simulink model "radio_FM_simulink_final"  (R2026b)
settings: Solver=FixedStepDiscrete  StopTime=0.6  FixedStep=sampling_time
values from neighbouring files (symbols this model uses):
  DC_fm = G_dem*fc_fm/df    [parametros.m]
  df = beta*B_fdm    (= 6000)    [parametros.m]
  epsilon = 1e-8    (= 1e-08)    [parametros.m]
  fc_am2 = 400    [parametros.m]
  fc_am3 = 800    [parametros.m]
  fc_fm = evalin('base','fc_fm')    [radio_gui.m]
  flo = f_rx + fi    [parametros.m]
  G_fdm = 1/(3*(1+mu))    (= 0.222222222222)    [parametros.m]
  K_am = pi/(G_fdm*mu) / (1 + (select == 1))    [parametros.m]
  Kdem = G_dem/(4*df)    (= 5.25945833333e-05)    [parametros.m]
  mu = 0.5    [parametros.m]
  sampling_time = 2e-6    (= 2e-06)    [parametros.m]
  select = evalin('base','select')    [radio_gui.m]
  Ts_d = M*sampling_time    (= 1e-05)    [parametros.m]
undefined symbols (not defined in the file or in its folder): dfilt, DiscIntNeverNeededParam
libraries: dsparch4 x6, simulink x2, dspfdesign x2
settings Model: Creator=henao  LastModifiedBy=henao
settings DataIOCC: SaveOutput=off  SignalLogging=off

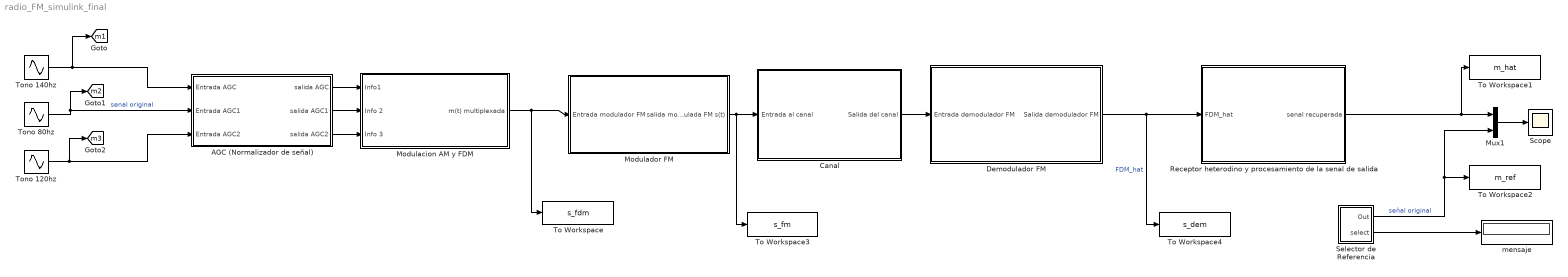
== system radio_FM_simulink_final ==
  AGC (Normalizador de señal) : Subsystem
  Canal : Subsystem
  Demodulador FM : Subsystem
  Modulacion AM y FDM : Subsystem
  Modulador FM : Subsystem
  Mux1 : Mux  Inputs=2
  Receptor heterodino y procesamiento de la senal de salida : Subsystem
  Scope : Scope
      settings: ActiveDisplayYMinimum=-1.3000748923673051  ActiveDisplayYMaximum=1.4483911176707998
  Selector de Referencia : Subsystem
  To Workspace : ToWorkspace  VariableName=s_fdm  SampleTime=-1
  To Workspace1 : ToWorkspace  VariableName=m_hat  SampleTime=-1
  To Workspace2 : ToWorkspace  VariableName=m_ref  SampleTime=-1
  To Workspace3 : ToWorkspace  VariableName=s_fm  SampleTime=-1
  To Workspace4 : ToWorkspace  VariableName=s_dem  SampleTime=-1
  Tono 120hz : Sin  Frequency=120*2*pi  SampleTime=sampling_time
  Tono 140hz : Sin  Amplitude=2  Frequency=140*2*pi  SampleTime=sampling_time
  Tono 80hz : Sin  Amplitude=3  Frequency=80*2*pi  SampleTime=sampling_time
  mensaje : Display
  tag scope: m1=global, m2=global, m3=global
  wires:
  Tono 80hz/1 -> AGC (Normalizador de señal)/2(Entrada AGC1), [m2]  "senal original"
  Tono 120hz/1 -> AGC (Normalizador de señal)/3(Entrada AGC2), [m3]
  Tono 140hz/1 -> AGC (Normalizador de señal)/1(Entrada AGC), [m1]
  AGC (Normalizador de señal)/1(salida AGC) -> Modulacion AM y FDM/1(Info1)
  AGC (Normalizador de señal)/2(salida AGC1) -> Modulacion AM y FDM/2(Info 2)
  AGC (Normalizador de señal)/3(salida AGC2) -> Modulacion AM y FDM/3(Info 3)
  Modulador FM/1(salida modulada FM s(t)) -> To Workspace3/1, Canal/1(Entrada al canal)
  Canal/1(Salida del canal) -> Demodulador FM/1(Entrada demodulador FM)
  Receptor heterodino y procesamiento de la senal de salida/1(senal recuperada) -> To Workspace1/1, Mux1/1
  Mux1/1 -> Scope/1
  Demodulador FM/1(Salida demodulador FM) -> To Workspace4/1, Receptor heterodino y procesamiento de la senal de salida/1(FDM_hat)  "FDM_hat"
  Selector de Referencia/1(Out) -> To Workspace2/1, Mux1/2  "señal original"
  Modulacion AM y FDM/1("m(t) multiplexada ") -> To Workspace/1, Modulador FM/1(Entrada modulador FM)
  Selector de Referencia/2(select) -> mensaje/1

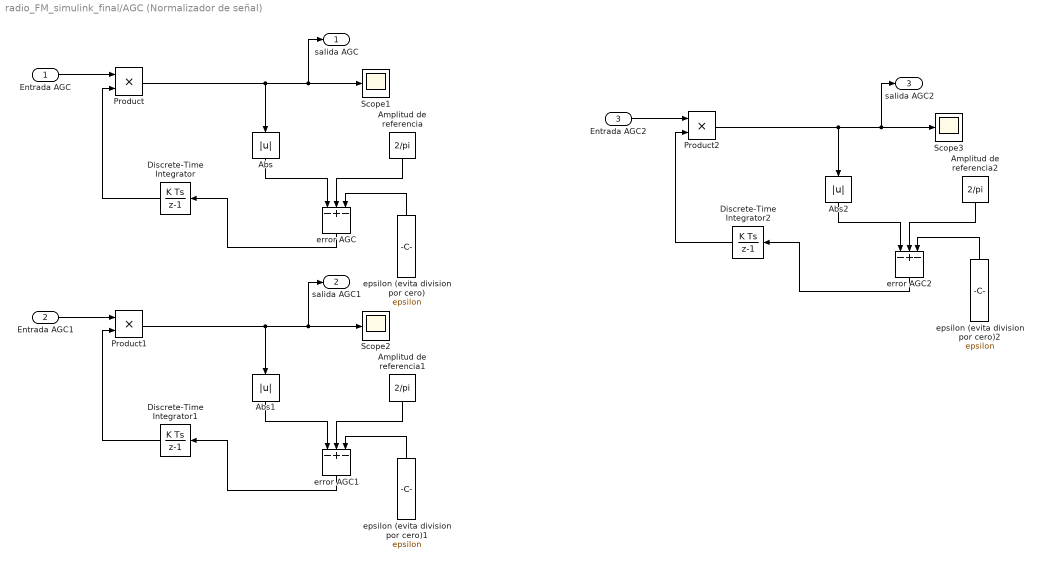
== system radio_FM_simulink_final/AGC (Normalizador de señal) ==
  Entrada AGC : Inport
  Entrada AGC1 : Inport  Port=2
  Entrada AGC2 : Inport  Port=3
  Abs : Abs  SaturateOnIntegerOverflow=off
  Abs1 : Abs  SaturateOnIntegerOverflow=off
  Abs2 : Abs  SaturateOnIntegerOverflow=off
  Amplitud de referencia : Constant  Value=2/pi
  Amplitud de referencia1 : Constant  Value=2/pi
  Amplitud de referencia2 : Constant  Value=2/pi
  Discrete-Time Integrator : DiscreteIntegrator  gainval=10  SampleTime=sampling_time  ICPrevOutput=DiscIntNeverNeededParam  ICPrevScaledInput=DiscIntNeverNeededParam
  Discrete-Time Integrator1 : DiscreteIntegrator  gainval=10  SampleTime=sampling_time  ICPrevOutput=DiscIntNeverNeededParam  ICPrevScaledInput=DiscIntNeverNeededParam
  Discrete-Time Integrator2 : DiscreteIntegrator  gainval=10  SampleTime=sampling_time  ICPrevOutput=DiscIntNeverNeededParam  ICPrevScaledInput=DiscIntNeverNeededParam
  Product : Product
  Product1 : Product
  Product2 : Product
  Scope1 : Scope
      settings: ActiveDisplayYMinimum=-1.05206  ActiveDisplayYMaximum=1.11653  DataLoggingVariableName=ScopeData3
  Scope2 : Scope
      settings: ActiveDisplayYMinimum=-1.05206  ActiveDisplayYMaximum=1.11653  DataLoggingVariableName=ScopeData2
  Scope3 : Scope
      settings: ActiveDisplayYMinimum=-1.05206  ActiveDisplayYMaximum=1.11653  DataLoggingVariableName=ScopeData4
  epsilon (evita division por cero) : Constant  Value=epsilon
  epsilon (evita division por cero)1 : Constant  Value=epsilon
  epsilon (evita division por cero)2 : Constant  Value=epsilon
  error AGC : Sum  Inputs=-+-
  error AGC1 : Sum  Inputs=-+-
  error AGC2 : Sum  Inputs=-+-
  salida AGC : Outport
  salida AGC1 : Outport  Port=2
  salida AGC2 : Outport  Port=3
  wires:
  error AGC/1 -> Discrete-Time Integrator/1
  Product/1 -> Abs/1, salida AGC/1, Scope1/1
  Abs/1 -> error AGC/1
  Amplitud de referencia/1 -> error AGC/2
  epsilon (evita division por cero)/1 -> error AGC/3
  Discrete-Time Integrator/1 -> Product/2
  Entrada AGC/1 -> Product/1
  Abs1/1 -> error AGC1/1
  Product1/1 -> Abs1/1, salida AGC1/1, Scope2/1
  epsilon (evita division por cero)1/1 -> error AGC1/3
  Entrada AGC1/1 -> Product1/1
  Amplitud de referencia1/1 -> error AGC1/2
  Discrete-Time Integrator1/1 -> Product1/2
  error AGC1/1 -> Discrete-Time Integrator1/1
  epsilon (evita division por cero)2/1 -> error AGC2/3
  error AGC2/1 -> Discrete-Time Integrator2/1
  Amplitud de referencia2/1 -> error AGC2/2
  Product2/1 -> Abs2/1, salida AGC2/1, Scope3/1
  Entrada AGC2/1 -> Product2/1
  Abs2/1 -> error AGC2/1
  Discrete-Time Integrator2/1 -> Product2/2

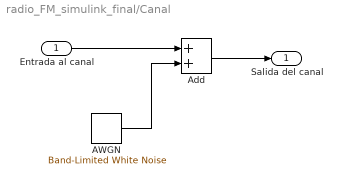
== system radio_FM_simulink_final/Canal ==
  Entrada al canal : Inport
  AWGN : simulink/Sources/Band-Limited White Noise  Cov=sigma2  Ts=sampling_time  seed=seed_ruido
  Add : Sum
  Salida del canal : Outport
  wires:
  Add/1 -> Salida del canal/1
  Entrada al canal/1 -> Add/1
  AWGN/1 -> Add/2

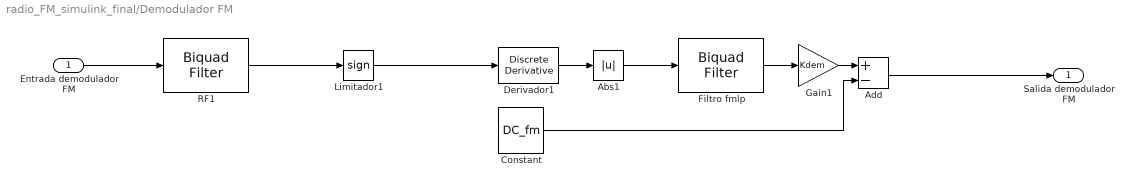
== system radio_FM_simulink_final/Demodulador FM ==
  Entrada demodulador FM : Inport
  Abs1 : Abs  SaturateOnIntegerOverflow=off
  Add : Sum  Inputs=+-
  Constant : Constant  Value=DC_fm
  Derivador1 : simulink/Discrete/Discrete Derivative  gainval=1  ICPrevScaledInput=0.0  OutMin=[]  OutMax=[]  OutDataType=fixdt(1, 16)  OutScaling=2^-10  DoSatur=off
  Filtro fmlp : dsparch4/Biquad Filter  FilterSource=Dialog parameters  CoeffSource=Specify via dialog  FilterObject=dfilt.df2tsos([1 0.3 0.4],[1 0.1 0.2])  IIRFiltStruct=Direct form II transposed  BiQuadCoeffs=sos_fmlp  ScaleValues=1  IC=0  ICnum=0  ICden=0  a0Flag=Warning  optimizeScaleValues=on  ScaleValueMode=Specify via input port (g)  roundingMode=Floor  overflowMode=off  scaleValueFracLength=14  denProdOutputFracLength=30  denAccumFracLength=30  secondMemoryFracLength=15
      settings: LibrarySourceBlock=dsphdlsupportfiltering/Biquad Filter
  Gain1 : Gain  Gain=Kdem
  Limitador1 : Signum
  RF1 : dsparch4/Biquad Filter  FilterSource=Dialog parameters  CoeffSource=Specify via dialog  FilterObject=dfilt.df2tsos([1 0.3 0.4],[1 0.1 0.2])  IIRFiltStruct=Direct form II transposed  BiQuadCoeffs=sos_rf  ScaleValues=1  IC=0  ICnum=0  ICden=0  a0Flag=Warning  optimizeScaleValues=on  ScaleValueMode=Specify via input port (g)  roundingMode=Floor  overflowMode=off  scaleValueFracLength=14  denProdOutputFracLength=30  denAccumFracLength=30  secondMemoryFracLength=15
      settings: LibrarySourceBlock=dsphdlsupportfiltering/Biquad Filter
  Salida demodulador FM : Outport
  wires:
  Entrada demodulador FM/1 -> RF1/1
  Filtro fmlp/1 -> Gain1/1
  Abs1/1 -> Filtro fmlp/1
  Derivador1/1 -> Abs1/1
  Limitador1/1 -> Derivador1/1
  RF1/1 -> Limitador1/1
  Add/1 -> Salida demodulador FM/1
  Gain1/1 -> Add/1
  Constant/1 -> Add/2

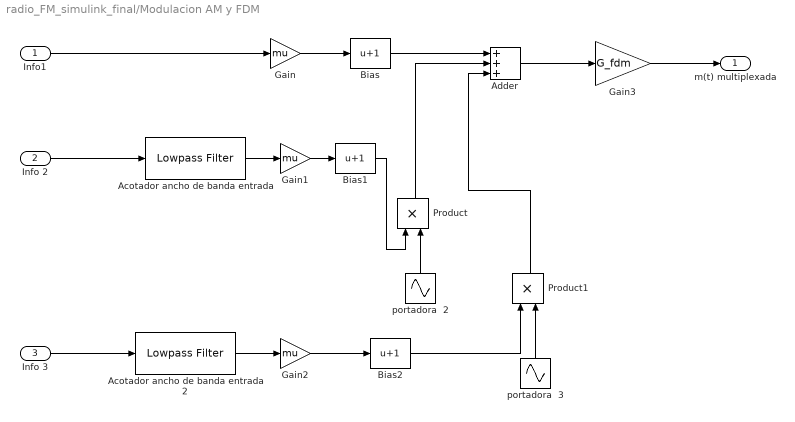
== system radio_FM_simulink_final/Modulacion AM y FDM ==
  Info1 : Inport
  Info 2 : Inport  Port=2
  Info 3 : Inport  Port=3
  Acotador ancho de banda entrada : dspfdesign/Lowpass Filter  FilterType=IIR  DesignForMinimumOrder=on  FilterOrder=50  PassbandFrequency=fp_in  StopbandFrequency=fs_in  PassbandRipple=Ap_in  StopbandAttenuation=As_in  SampleRateMode=Specify on dialog  SampleRate=sampling_frec  SimulateUsing=Interpreted execution  roundingMode=Floor  coeffsDataTypeStr=fixdt(1,16)
  Acotador ancho de banda entrada 2 : dspfdesign/Lowpass Filter  FilterType=IIR  DesignForMinimumOrder=on  FilterOrder=50  PassbandFrequency=fp_in  StopbandFrequency=fs_in  PassbandRipple=Ap_in  StopbandAttenuation=As_in  SampleRateMode=Specify on dialog  SampleRate=sampling_frec  SimulateUsing=Interpreted execution  roundingMode=Floor  coeffsDataTypeStr=fixdt(1,16)
  Adder : Sum  Inputs=+++
  Bias : Bias  Bias=1  SaturateOnIntegerOverflow=off
  Bias1 : Bias  Bias=1  SaturateOnIntegerOverflow=off
  Bias2 : Bias  Bias=1  SaturateOnIntegerOverflow=off
  Gain : Gain  Gain=mu
  Gain1 : Gain  Gain=mu
  Gain2 : Gain  Gain=mu
  Gain3 : Gain  Gain=G_fdm
  Product : Product
  Product1 : Product
  portadora  2 : Sin  Frequency=2*pi*fc_am2  Phase=pi/2  SampleTime=sampling_time
  portadora  3 : Sin  Frequency=2*pi*fc_am3  Phase=pi/2  SampleTime=sampling_time
  "m(t) multiplexada " : Outport
  wires:
  portadora  3/1 -> Product1/2
  portadora  2/1 -> Product/2
  Info 2/1 -> Acotador ancho de banda entrada/1
  Info 3/1 -> Acotador ancho de banda entrada 2/1
  Adder/1 -> Gain3/1
  Info1/1 -> Gain/1
  Gain/1 -> Bias/1
  Bias/1 -> Adder/1
  Product1/1 -> Adder/3
  Product/1 -> Adder/2
  Gain3/1 -> "m(t) multiplexada "/1
  Gain1/1 -> Bias1/1
  Acotador ancho de banda entrada/1 -> Gain1/1
  Bias1/1 -> Product/1
  Gain2/1 -> Bias2/1
  Acotador ancho de banda entrada 2/1 -> Gain2/1
  Bias2/1 -> Product1/1

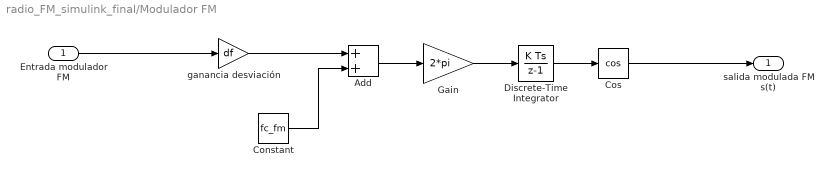
== system radio_FM_simulink_final/Modulador FM ==
  Entrada modulador FM : Inport
  Add : Sum
  Constant : Constant  Value=fc_fm  SampleTime=sampling_time
  Cos : Trigonometry  Operator=cos
  Discrete-Time Integrator : DiscreteIntegrator  gainval=1  SampleTime=sampling_time  ICPrevOutput=DiscIntNeverNeededParam  ICPrevScaledInput=DiscIntNeverNeededParam
  Gain : Gain  Gain=2*pi
  ganancia desviación : Gain  Gain=df
  salida modulada FM s(t) : Outport
  wires:
  Discrete-Time Integrator/1 -> Cos/1
  Entrada modulador FM/1 -> ganancia desviación/1
  Cos/1 -> salida modulada FM s(t)/1
  Constant/1 -> Add/2
  Add/1 -> Gain/1
  ganancia desviación/1 -> Add/1
  Gain/1 -> Discrete-Time Integrator/1

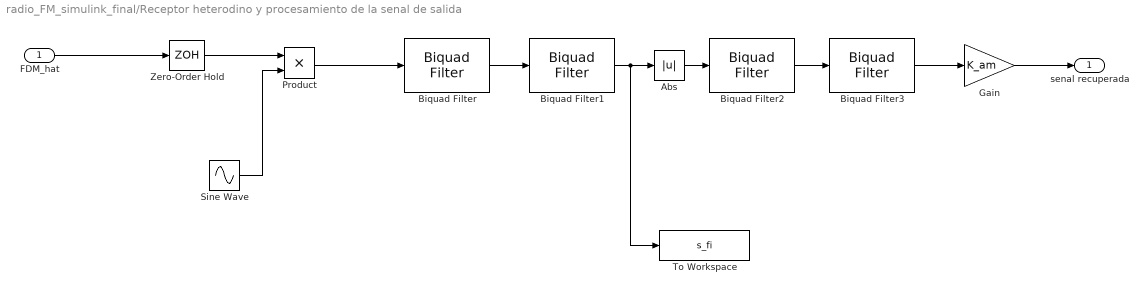
== system radio_FM_simulink_final/Receptor heterodino y procesamiento de la senal de salida ==
  FDM_hat : Inport
  Abs : Abs  SaturateOnIntegerOverflow=off
  Biquad Filter : dsparch4/Biquad Filter  FilterSource=Dialog parameters  CoeffSource=Specify via dialog  FilterObject=BQF  IIRFiltStruct=Direct form II transposed  BiQuadCoeffs=sos_lp1  ScaleValues=1  IC=0  ICnum=0  ICden=0  a0Flag=Warning  optimizeScaleValues=on  ScaleValueMode=Specify via input port (g)  InputProcessing=Columns as channels (frame based)  roundingMode=Floor  overflowMode=off  scaleValueFracLength=14  denProdOutputFracLength=30  denAccumFracLength=30  secondMemoryFracLength=15
  Biquad Filter1 : dsparch4/Biquad Filter  FilterSource=Dialog parameters  CoeffSource=Specify via dialog  FilterObject=BQF  IIRFiltStruct=Direct form II transposed  BiQuadCoeffs=sos_fi  ScaleValues=1  IC=0  ICnum=0  ICden=0  a0Flag=Warning  optimizeScaleValues=on  ScaleValueMode=Specify via input port (g)  InputProcessing=Columns as channels (frame based)  roundingMode=Floor  overflowMode=off  scaleValueFracLength=14  denProdOutputFracLength=30  denAccumFracLength=30  secondMemoryFracLength=15
  Biquad Filter2 : dsparch4/Biquad Filter  FilterSource=Dialog parameters  CoeffSource=Specify via dialog  FilterObject=BQF  IIRFiltStruct=Direct form II transposed  BiQuadCoeffs=sos_aud  ScaleValues=1  IC=0  ICnum=0  ICden=0  a0Flag=Warning  optimizeScaleValues=on  ScaleValueMode=Specify via input port (g)  InputProcessing=Columns as channels (frame based)  roundingMode=Floor  overflowMode=off  scaleValueFracLength=14  denProdOutputFracLength=30  denAccumFracLength=30  secondMemoryFracLength=15
  Biquad Filter3 : dsparch4/Biquad Filter  FilterSource=Dialog parameters  CoeffSource=Specify via dialog  FilterObject=BQF  IIRFiltStruct=Direct form II transposed  BiQuadCoeffs=sos_dc  ScaleValues=1  IC=0  ICnum=0  ICden=0  a0Flag=Warning  optimizeScaleValues=on  ScaleValueMode=Specify via input port (g)  InputProcessing=Columns as channels (frame based)  roundingMode=Floor  overflowMode=off  scaleValueFracLength=14  denProdOutputFracLength=30  denAccumFracLength=30  secondMemoryFracLength=15
  Gain : Gain  Gain=K_am
  Product : Product
  Sine Wave : Sin  Frequency=2*pi*flo  Phase=pi/2  SampleTime=Ts_d
  To Workspace : ToWorkspace  VariableName=s_fi  SampleTime=-1
  Zero-Order Hold : ZeroOrderHold  SampleTime=Ts_d
  senal recuperada : Outport
  wires:
  Biquad Filter2/1 -> Biquad Filter3/1
  Sine Wave/1 -> Product/2
  Biquad Filter/1 -> Biquad Filter1/1
  Abs/1 -> Biquad Filter2/1
  Biquad Filter3/1 -> Gain/1
  Biquad Filter1/1 -> To Workspace/1, Abs/1
  Zero-Order Hold/1 -> Product/1
  Gain/1 -> senal recuperada/1
  FDM_hat/1 -> Zero-Order Hold/1
  Product/1 -> Biquad Filter/1

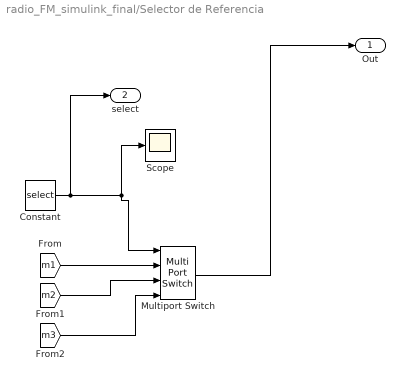
== system radio_FM_simulink_final/Selector de Referencia ==
  Constant : Constant  Value=select
  Multiport Switch : MultiPortSwitch  SaturateOnIntegerOverflow=off  InputSameDT=off
  Scope : Scope
      settings: ActiveDisplayYMinimum=2  ActiveDisplayYMaximum=4
  Out : Outport
  select : Outport  Port=2
  wires:
  [m1] -> Multiport Switch/2
  Constant/1 -> select/1, Multiport Switch/1, Scope/1
  Multiport Switch/1 -> Out/1
  [m2] -> Multiport Switch/3
  [m3] -> Multiport Switch/4
